simulink model "sschdlexBridgeRectifierModel"  (R2026a)
settings: Solver=FixedStepDiscrete  StopTime=0.05  MaxStep=1e-3  AbsTol=1e-4
PreLoadFcn:
  | Ts_FPGA = 1e-6; % FPGA sample time
  | Ts_CPU = 1e-6; % CPU sample time
  | Vf = 0.6; % Diode Forward Voltage
  | Ron = 0.3; % Diode On-state resistance
  | Goff = 1e-8; % Diode Off-state conductance
  | Ls = 1e-6; % Source Inductance
  | Rs = 0.01; % Source Resistance
  | C = 1e-3; % Load Capacitor
  | R = 20; % Load resistance
libraries: fl_lib x6, ee_lib x6, nesl_utility x4
CloseFcn:
  | clear all;
settings Model: DataTypeOverride=Off  Creator=The MathWorks, Inc.  LastModifiedBy=The MathWorks, Inc.
settings OptimizationCC: ConditionallyExecuteInputs=off  InheritOutputTypeSmallerThanSingle=on
settings DebuggingCC: ArtificialAlgebraicLoopMsg=error  MultiTaskDSMMsg=warning  MultiTaskCondExecSysMsg=none  SingleTaskRateTransMsg=error  PregeneratedLibrarySubsystemCodeDiagnostic=none
settings HardwareCC: ProdHWDeviceType=ASIC/FPGA->ASIC/FPGA  TargetBitPerLong=64.0  TargetBitPerPointer=64.0  TargetBitPerSizeT=64.0  TargetBitPerPtrDiffT=64.0  TargetLongLongMode=on  TargetIntDivRoundTo=Zero  TargetEndianess=LittleEndian  TargetWordSize=64.0  TargetHWDeviceType=Custom Processor->MATLAB Host Computer  ProdEqTarget=off
settings ModelReferenceCC: ModelReferenceNumInstancesAllowed=Single
settings SimscapeCC: SimscapeNormalizeSystem=off  SimscapeNominalValues="[{\"value\":\"10\",\"unit\":\"V\"},{\"value\":\"1\",\"unit\":\"A\"},{\"value\":\"10\",\"unit\":\"N*m\"},{\"value\":\"10\",\"unit\":\"bar\"},{\"value\":\"100\",\"unit\":\"kJ/kg\"},{\"value\":\"1\",\"unit\":\"kW\"},{\"value\":\"300\",\"unit\":\"K\"},{\"value\":\"100\",\"unit\":\"cm^3/s\"},{\"value\":\"1\",\"unit\":\"kN\"},{\"value\":\"1\",\"unit\":\"g/cm^3\"},{\"value\":\"1\",\"unit\":\"l\"},{\"value\":\"1\",\"unit\":\"cm^2\"},{\"value\":\"60\",\"unit\":\"Hz\"}]"  SimscapeLogType=none  SimscapeLogSimulationStatistics=on  SimscapeLogLimitData=off  SimscapeLogDataHistory=5000.0

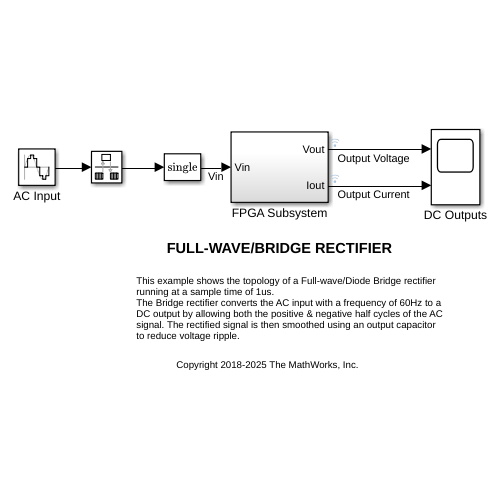
[thumbnail: Simulink's stored preview of the top-level diagram]
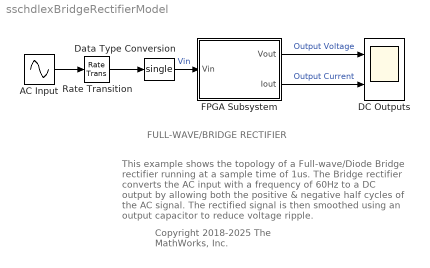
== system sschdlexBridgeRectifierModel ==
  note: FULL-WAVE/BRIDGE RECTIFIER
  note: This example shows the topology of a Full-wave/Diode Bridge rectifier running at a sample time of 1us.
      | The Bridge rectifier converts the AC input with a frequency of 60Hz to a DC output by allowing both the positive & negative half cycles of the AC signal. The rectified signal is then smoothed using an output capacitor to reduce voltage ripple.
  note: Copyright 2018-2025 The MathWorks, Inc.
  AC Input : Sin  Amplitude=100  Frequency=2*pi*60  SampleTime=Ts_CPU
  DC Outputs : Scope  NumInputPorts=2
      settings: ActiveDisplayYMinimum=-11.721594810485838  ActiveDisplayYMaximum=105.49435329437256
  Data Type Conversion : DataTypeConversion  OutDataTypeStr=single  SaturateOnIntegerOverflow=off  RndMeth=Floor
  FPGA Subsystem : Subsystem
  Rate Transition : RateTransition
  wires:
  FPGA Subsystem/1(Vout) -> DC Outputs/1  "Output Voltage"
  FPGA Subsystem/2(Iout) -> DC Outputs/2  "Output Current"
  Rate Transition/1 -> Data Type Conversion/1
  AC Input/1 -> Rate Transition/1
  Data Type Conversion/1 -> FPGA Subsystem/1(Vin)  "Vin"

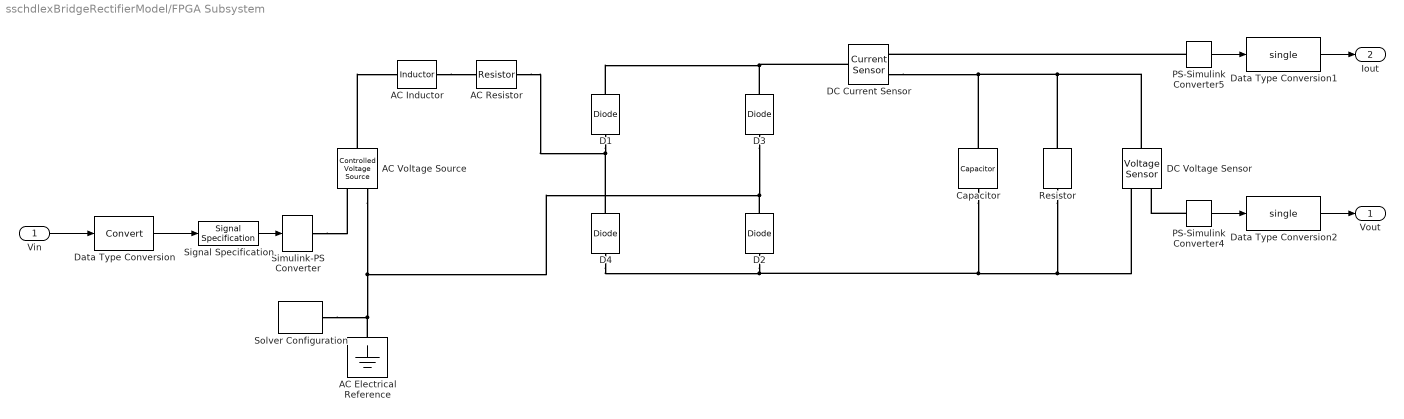
== system sschdlexBridgeRectifierModel/FPGA Subsystem ==
  Vin : Inport
  AC Electrical Reference : fl_lib/Electrical/Electrical Elements/Electrical Reference
  AC Inductor : fl_lib/Electrical/Electrical Elements/Inductor  l=Ls H  r=0 Ohm  g=0 1/Ohm  i_specify=off  i_priority=High  i=0 A  i_nominal_specify=off  i_nominal_value=1  i_nominal_unit=A  v_specify=off  v_priority=High  v=0 V  v_nominal_specify=off  v_nominal_value=1  v_nominal_unit=V  i_L_specify=on  i_L_priority=High  i_L=0 A  i_L_nominal_specify=off  i_L_nominal_value=1  i_L_nominal_unit=A
  AC Resistor : fl_lib/Electrical/Electrical Elements/Resistor  R=Rs Ohm  i_specify=off  i_priority=High  i=0 A  i_nominal_specify=off  i_nominal_value=1  i_nominal_unit=A  v_specify=off  v_priority=High  v=0 V  v_nominal_specify=off  v_nominal_value=1  v_nominal_unit=V
  AC Voltage Source : fl_lib/Electrical/Electrical Sources/Controlled Voltage Source
  Capacitor : ee_lib/Passive/Capacitor  cap_option=ee.enum.passive.capacitor.capOption.const  c=C F  Cvec=[1e-05, 1e-06] F  Vvec=[0, 10] V  CV_table_symmetry=1  f_vec=[1, 10] kHz  DFext_vec=[.8, 1.2]  enable_C_tol=0  averaging_period=0 s  C_tol=5  tol_distribution=1  nSigma=4  r=1e-6 Ohm  g=0 1/Ohm  enable_operating_limits=0  operating_limit_action=2  max_working_voltage_range=[-25, 25] V  power_rating=1 W  maxTemperature=85 degC  thermalEnable=false  thermalMass=1 J/K  i_specify=off  i_priority=None  i=0 A  i_nominal_specify=off  i_nominal_value=1  i_nominal_unit=A  v_specify=off  v_priority=None  v=0 V  v_nominal_specify=off  v_nominal_value=1  v_nominal_unit=V  vc_specify=off  vc_priority=High  vc=0 V  vc_nominal_specify=off  vc_nominal_value=1  vc_nominal_unit=V  T_specify=off  T_priority=None  T=298.15 K  T_nominal_specify=off  T_nominal_value=1  T_nominal_unit=K
  D{1..4} (4 alike) : ee_lib/Semiconductors & Converters/Diode  ModelType=ee.enum.diode.modelType.pwl  TableType=ee.enum.diode.tableType.IfMat  IfMat=[.07, .12, .19, 1.75, 4.24, 7.32, 11.2; .16, .3, .72, 2.14, 5.02, 8.35, 13.12] A  VfMat=[.9, 1.15, 1.25, 1.5, 1.75, 2.17, 2.6, 2.85; .58, .68, .75, 1.1, 1.38, 1.77, 2.27, 2.7] V  TjVec=[25, 125] degC  VfVec=[.5, .7, .9, 1.3, 1.7, 2.1, 2.5] V  IfVec=[.1, .2, .5, 1, 2, 4, 7, 10] A  IrMat=[1e-06, 2e-06, 5e-06, 1e-05, 2.5e-05, 5e-05, .0001; 2e-06, 5e-06, 1e-05, 4e-05, 8e-05, .0002, .0005] A  VrMat=[10, 100, 200, 250, 300, 325, 350; 10, 70, 160, 220, 270, 300, 320] V  VrVec=[10, 20, 40, 50, 70, 80, 100] V  IrVec=[1e-06, 2e-06, 5e-06, 1e-05, 2e-05, 5e-05, .0001] A  Vf=Vf V  Ron=Ron Ohm  Goff=Goff S  prmExp=ee.enum.diode.expParam.useTwo  I12=[.0137, .545] A  V12=[.6, .7] V  RS=0 Ohm  Tmeas=25 degC  IS=1e-12 A  ec=1  I1=0.0137 A  V1=0.6 V  N_series=1  N_parallel=1  ZenerEnable=false  Rz=0.3 Ohm  BV=inf V  C_param=ee.enum.diode.capParam.fixed  CJ=0 pF  CJ0=5 pF  Vvec=[.1, 10, 100] V  Cvec=[3.5, 1, .4] pF  VJ=1 V  Mgrad=0.5  FC=0.5  Q_param=ee.enum.diode.recoveryParam.off  iRM=-7.15 A  iF=4 A  didt=-750 A/us  trr_factor=3  trr=115 ns  Qrr=150 nA*s  Vr=-600 V  Ls=150 nH  Erec=0.03 J  TT=50 ns  tau=100 ns  T_param=ee.enum.diode.temperatureParam.off  Tdevice=25 degC  I1_T2=0.245 A  V1_T2=0.5 V  IS_T2=1.25e-7 A  Tmeas2=125 degC  XTI_param=ee.enum.diode.xtiParam.pn  XTI=3  EG_param=ee.enum.diode.egapParam.material_si  EG=1.11 eV  dBVdT=0 V/K  enable_fault_input=simscape.enum.onoff.off  i_specify=off  i_priority=None  i=0 A  i_nominal_specify=off  i_nominal_value=1  i_nominal_unit=A  v_specify=off  v_priority=None  v=0 V  v_nominal_specify=off  v_nominal_value=1  v_nominal_unit=V  v_capacitor_specify=off  v_capacitor_priority=None  v_capacitor=0 V  v_capacitor_nominal_specify=off  v_capacitor_nominal_value=1  v_capacitor_nominal_unit=V  Qj_specify=off  Qj_priority=High  Qj=0 C  Qj_nominal_specify=off  Qj_nominal_value=1  Qj_nominal_unit=C  i_diode_specify=off  i_diode_priority=None  i_diode=0 A  i_diode_nominal_specify=off  i_diode_nominal_value=1  i_diode_nominal_unit=A  v_diode_specify=off  v_diode_priority=None  v_diode=0 V  v_diode_nominal_specify=off  v_diode_nominal_value=1  v_diode_nominal_unit=V  i_capacitor_specify=off  i_capacitor_priority=None  i_capacitor=0 A  i_capacitor_nominal_specify=off  i_capacitor_nominal_value=1  i_capacitor_nominal_unit=A  fidelity_level=ee.enum.diode.fidelity.includeChargeDyn  rec_loss_model=ee.enum.diode.reverseRecoveryModel.fixed  ErecVal=0 J  scaleWithIandV=true  ErecMat=zeros(2, 3) J  ErecMat3D=zeros(2, 3, 2) J  TjrecVec=[298.15, 398.15] K  IfrecVec=[.1, 1, 10] A  IrecVal=10 A  VrecVal=10 V  VrecVec=[0, 100] V  tFilter=1 / 1000 / 100 s  thermal_network_parameterization=ee.enum.thermalNetworkTopology.junctionCase  Rth=[0, 10] K/W  Rth_Cauer=[1, 3, 10] K/W  Rth_Foster=[4, 6] K/W  thermal_mass_parameterization=ee.enum.thermalNetwork.timeconstant  thermal_mass=[0, 1] J/K  thermal_mass_Cauer=[.1, .3, 1] J/K  thermal_mass_Foster=[1.5, 3] J/K  thermal_time_constant=[0, 10] s  thermal_time_constant_Cauer=[1, 3, 10] s  thermal_time_constant_Foster=[6, 18] s  thermal_mass_initial_temperatures=[25, 25] degC  thermal_mass_initial_temperatures_Cauer=[25, 25, 25] degC  junction_thermal_mass=0.01 J/K  Tvec_initial_Foster=[25, 25, 25, 25] degC  no_thermal_network=0  junction_temperature_specify=off  junction_temperature_priority=None  junction_temperature=25 degC  junction_temperature_nominal_specify=off  junction_temperature_nominal_value=1  junction_temperature_nominal_unit=degC
  DC Current Sensor : fl_lib/Electrical/Electrical Sensors/Current Sensor
  DC Voltage Sensor : fl_lib/Electrical/Electrical Sensors/Voltage Sensor
  Data Type Conversion : DataTypeConversion  SaturateOnIntegerOverflow=off  RndMeth=Floor
  Data Type Conversion1 : DataTypeConversion  OutDataTypeStr=single  SaturateOnIntegerOverflow=off  RndMeth=Floor
  Data Type Conversion2 : DataTypeConversion  OutDataTypeStr=single  SaturateOnIntegerOverflow=off  RndMeth=Floor
  PS-Simulink Converter4 : nesl_utility/PS-Simulink Converter  PhysicalDomain=network_engine_domain  SubClassName=ps_output  LeftPortType=input  RightPortType=output  PseudoPeriodic=off  Frequencies=[]  VectorFormat=1-D array  Unit=1  AffineConversion=off
  PS-Simulink Converter5 : nesl_utility/PS-Simulink Converter  PhysicalDomain=network_engine_domain  SubClassName=ps_output  LeftPortType=input  RightPortType=output  PseudoPeriodic=off  Frequencies=[]  VectorFormat=1-D array  Unit=1  AffineConversion=off
  Resistor : ee_lib/Passive/Resistor  R=R Ohm  enable_R_tol=0  R_tol=5  tol_distribution=1  nSigma=4  enable_operating_limits=0  operating_limit_action=2  power_rating=1 W  max_working_voltage=100 V  noise_mode=0  Tdevice=25 degC  sample_time=1e-3 s  repeatability=1  user_seed=0  auto_seed=659950577  power_derating_T1=70 degC  power_derating_T2=155 degC  operating_temperature_range_vec=[-50, 150] degC  alpha=3.93e-3 1/K  Tmeas=25 degC  thermal_mass=100 J/K  temperature_specify=off  temperature_priority=High  temperature=298.15 K  temperature_nominal_specify=off  temperature_nominal_value=1  temperature_nominal_unit=K
  Signal Specification : SignalSpecification  SampleTime=Ts_FPGA
  Simulink-PS Converter : nesl_utility/Simulink-PS Converter  PhysicalDomain=network_engine_domain  SubClassName=ps_input  LeftPortType=input  RightPortType=output  PseudoPeriodic=off  Frequencies=[]  NoiseDistribution=none  NoiseParameters=[]  Unit=1  AffineConversion=off  FilteringAndDerivatives=zero  SimscapeFilterOrder=1  InputFilterTimeConstant=0.001  UdotUserProvided=1
  Solver Configuration : nesl_utility/Solver Configuration  PhysicalDomain=network_engine_domain  SubClassName=solver  LeftPortType=input  RightPortType=generic  Tones=[]  Harmonics=[]  SimulateNoise=off  Profile=off  UseLocalSampling=off  EnableSwitchedLinearOptims=off  FrequencyDomain=off  UseCCode=off  RelTol=0.001  AbsTol=1e-06  MinStep=1e-09  ToWorkspace=off  RevertToSquareIcSolve=off  NumHomotopyIterations=100  PhasorMode=off  PhasorModeNumHarmonics=1  ConsistencySolver=NEWTON_FTOL  CanonicalOrdering=UNORDERED  OptimizeIntermediates=UNOPTIMIZED  IndexReductionMethod=DerivativeReplacement  DoDC=off  ResidualTolerance=1e-09  ConsistencyTolSource=GLOBAL  ConsistencyAbsTol=0.001  ConsistencyRelTol=0.001  ConsistencyTolFactor=0.001  UseLocalSolver=on  LocalSolverChoice=NE_BACKWARD_EULER_ADVANCER  ResolveIndetEquations=on  FunctionEvalNumThread=1  LocalSolverSampleTime=Ts_FPGA  DoFixedCost=off  MaxNonlinIter=2  MaxModeIter=2  ComputeImpulses=off  ImpulseIterations=2  LinearAlgebra=Sparse  LinearAlgebraNumThread=0  EquationFormulation=NE_TIME_EF  DelaysMemoryBudget=1024  AutomaticFiltering=on  FilteringTimeConstant=0.001  PartitionStorageMethod=AS_NEEDED  PartitionMemoryBudget=1024  PartitionMethod=FAST  MultibodyUseLocalSolver=off  MultibodyLocalSolverChoice=ODE1  MultibodyLocalSolverSampleTime=0.001
  Vout : Outport  VectorParamsAs1DForOutWhenUnconnected=off
  Iout : Outport  Port=2  VectorParamsAs1DForOutWhenUnconnected=off
  wires:
  PS-Simulink Converter4/1 -> Data Type Conversion2/1
  PS-Simulink Converter5/1 -> Data Type Conversion1/1
  Data Type Conversion/1 -> Signal Specification/1
  Vin/1 -> Data Type Conversion/1
  Signal Specification/1 -> Simulink-PS Converter/1
  Data Type Conversion1/1 -> Iout/1
  Data Type Conversion2/1 -> Vout/1
  connections:
  Capacitor/RConn1 -- DC Voltage Sensor/RConn2 -- Resistor/RConn1 -- D4/LConn1 -- D2/LConn1
  AC Electrical Reference/LConn1 -- AC Voltage Source/RConn2 -- D3/LConn1 -- D2/RConn1 -- Solver Configuration/RConn1
  D1/LConn1 -- D4/RConn1 -- AC Resistor/RConn1
  PS-Simulink Converter5/LConn1 -- DC Current Sensor/RConn1
  PS-Simulink Converter4/LConn1 -- DC Voltage Sensor/RConn1
  Simulink-PS Converter/RConn1 -- AC Voltage Source/RConn1
  D1/RConn1 -- DC Current Sensor/LConn1 -- D3/RConn1
  DC Voltage Sensor/LConn1 -- Resistor/LConn1 -- Capacitor/LConn1 -- DC Current Sensor/RConn2
  AC Inductor/RConn1 -- AC Resistor/LConn1
  AC Voltage Source/LConn1 -- AC Inductor/LConn1
